simulink model "SK_x46s"  (R2026a)
settings: Solver=ode14x  StopTime=p_T  FixedStep=p_Ts
undefined symbols (not defined in the file): dspblkCoreblockFVToolHelper, gcbh, isdone_init, p_base_mass, p_base_w, p_cmd_scale, p_cost_type, p_damp_scale, p_delay_steps, p_inertia_scale, p_j6_lim, p_lambda, p_obs_mode, p_obs_noise, p_q0, p_reward_mode, p_theta, p_Ts_agent, reward_init, X, Y, Z
libraries: sm_lib x98, nesl_utility x50, rllib x1, sharedutil x1
(part 3 of 3)

== matlab function SK_x46s/Obs Transform ==
  data: u input; y output; mode input; sigma input
function y = obs_transform(u, mode, sigma)
% mode 0: Beobachtung wie im Training [ep; ev; v_base; w_base; q; dq; e_ori]
% mode 1: wie Deploy-Skript V2.1 (Befund A22): Reihenfolge [ep; ev; q; dq; v_base; w_base; e_ori],
%         Vorzeichen Soll - Ist, Basisgroessen null, e_ori = Endeffektor-Orientierung, Clipping wie V2.1
% sigma: 29x1 Standardabweichungen fuer gaussches Beobachtungsrauschen (D7), 0 = kein Rauschen.
%        Das Rauschen kommt aus MATLAB (desktop_obs_randn), damit rng-Seeds wirken.
coder.extrinsic('desktop_v21_eori', 'desktop_obs_randn');
y = u;
if any(sigma > 0)
    nz = zeros(29, 1);
    nz = desktop_obs_randn();
    y = y + sigma .* nz;
end
if mode == 1
    q = y(13:19);
    dq = y(20:26);
    e = zeros(3, 1);
    e = desktop_v21_eori(q);
    y = [-y(1:3); -y(4:6); q; dq; zeros(3, 1); zeros(3, 1); e];
    qlo = [-2*pi; -2.41; -2*pi; -2.66; -2.23; -2.01; -2*pi];
    dqlim = [1.3963; 1.3963; 1.3963; 1.3963; 1.2218; 1.2218; 1.2218];
    hi = [0.5*ones(3,1); 1.0*ones(3,1); -qlo; dqlim; 0.5*ones(3,1); 1.0*ones(3,1); pi*ones(3,1)];
    y = min(max(y, -hi), hi);
end

== matlab function SK_x46s/Reward/MATLAB Function ==
  data: ep input; reward output; ev input; dq_cmd input; dq_cmd_prev input; isDone output; w_base input; e_ori input; cost output; p_reward_mode parameter; p_base_w parameter; p_lambda parameter; p_theta parameter; p_cost_type parameter
function [reward, isDone, cost] = rewardFcn(ep, ev, dq_cmd, dq_cmd_prev, w_base, e_ori, p_reward_mode, ...
p_base_w, p_lambda, p_theta, p_cost_type)
% Reward des Tracking-Trainings mit Varianten fuer D12 (Befund A51)
%   p_reward_mode 0: wie im Training seit 09.04. (Basis-Strafen und Basis-Bonus)
%                 1: ohne Basis-Terme, wie beim fruehen PPO (Modell im Commit 50ad2ce, ohne Abbruch bei ori > 1)
%                 2: wie 0, der Basis-Bonus gilt nur bei EE-Fehler < 5 cm
%                 3: dicht und gekoppelt: glatte EE-Boni, Basis-Bonus mit der Tracking-Guete gewichtet,
%                    linearer Positionsterm -5*min(|ep|, 0,2) (hoechstens -1 pro Schritt, damit ein Abbruch
%                    nicht billiger wird als Weiterfahren). Basis-Strafen wie 0
%                 4: wie 2, dazu auf der Bahn (EE-Fehler < 5 cm) ein glatter Basis-Term
%                    +p_base_w*exp(-(ori/0,05)^2), p_base_w = 2 in D16, variiert in D17
%                 5: wie 1 (nur Tracking), dazu -p_lambda*cost (Nebenbedingung auf die Basisdrehung, X1)
%   cost: Kosten der Nebenbedingung, in allen Modi berechnet. p_cost_type 1: 1 wenn ori > p_theta,
%         2: max(0, ori - p_theta)/p_theta. In Abbruchschritten 0
mode = p_reward_mode;
cost = 0;

if any(~isfinite([ep; ev; dq_cmd; dq_cmd_prev; w_base; e_ori]))
    reward = -50;
    isDone = true;
    return;
end

dist   = norm(ep);
vel    = norm(ev);
w_norm = norm(w_base);
ori    = norm(e_ori);

if dist > 0.5 || vel > 2.0 || (mode ~= 1 && mode ~= 5 && ori > 1.0)
    reward = -50;
    isDone = true;
    return;
end

c_pos = min(ep.' * ep, 0.25);
c_vel = min(ev.' * ev, 4.0);
c_u   = min(dq_cmd.' * dq_cmd, 10.0);
du    = dq_cmd - dq_cmd_prev;
c_du  = min(du.' * du, 10.0);
c_ori = min(e_ori.' * e_ori, 0.5);
c_w   = min(w_base.' * w_base, 1.0);

if p_cost_type == 2
    cost = max(0, ori - p_theta) / p_theta;
elseif ori > p_theta
    cost = 1;
end

if mode == 1 || mode == 5
    reward = - 20.0 * c_pos - 2.0 * c_vel - 0.02 * c_u - 0.05 * c_du;
else
    reward = ...
        - 20.0  * c_pos ...
        -  2.0  * c_vel ...
        -  0.02 * c_u   ...
        -  0.05 * c_du  ...
        -  8.0  * c_ori ...
        -  4.0  * c_w;
end

if mode == 3
    g = exp(-(dist / 0.05)^2);
    reward = reward - 5.0 * min(dist, 0.2) + 1.0 * g + 3.0 * exp(-(dist / 0.02)^2) ...
        + 2.0 * g * exp(-(ori / 0.02)^2) * exp(-(w_norm / 0.01)^2);
else
    if dist < 0.05
        reward = reward + 1;
    end
    if dist < 0.02
        reward = reward + 3;
    end
    if mode == 0 && ori < 0.02 && w_norm < 0.01
        reward = reward + 2;
    end
    if mode == 2 && ori < 0.02 && w_norm < 0.01 && dist < 0.05
        reward = reward + 2;
    end
    if mode == 4 && dist < 0.05
        reward = reward + p_base_w * exp(-(ori / 0.05)^2);
        if ori < 0.02 && w_norm < 0.01
            reward = reward + 2;
        end
    end
end
if mode == 5
    reward = reward - p_lambda * cost;
end

isDone = false;
end

== matlab function SK_x46s/Robot/Impuls Monitor/MATLAB Function ==
  data: v1 input; p_tot output; w1 input; q1 input; v2 input; w2 input; q2 input; v3 input; w3 input; q3 input; v4 input; w4 input; q4 input; v5 input; w5 input; q5 input
function p_tot = totalMomentum( ...
    v1,w1,q1, ...
    v2,w2,q2, ...
    v3,w3,q3, ...
    v4,w4,q4, ...
    v5,w5,q5)

%#codegen

    % Massen
    m = [5; 1; 1; 1; 1];

    % COM-Offsets im jeweiligen Link-Frame
    r_link = [ 0.0  0.0  0.0;   % Link 1
               0.5  0.0  0.0;   % Link 2
               0.5  0.0  0.0;   % Link 3
               0.5  0.0  0.0;   % Link 4
               0.5  0.0  0.0];  % Link 5

    % Initialisiere Gesamtimpuls
    p_tot = zeros(3,1);

    % Link 1
    p_tot = p_tot + linkMomentum(v1, w1, q1, m(1), r_link(1,:).');

    % Link 2
    p_tot = p_tot + linkMomentum(v2, w2, q2, m(2), r_link(2,:).');

    % Link 3
    p_tot = p_tot + linkMomentum(v3, w3, q3, m(3), r_link(3,:).');

    % Link 4
    p_tot = p_tot + linkMomentum(v4, w4, q4, m(4), r_link(4,:).');

    % Link 5
    p_tot = p_tot + linkMomentum(v5, w5, q5, m(5), r_link(5,:).');

end

function p = linkMomentum(v, w, q, m, r_link)
% v, w: 3x1 im World-Frame
% q: 4x1 Quaternion [w x y z], Orientierung Link relativ zu World
% r_link: 3x1 COM-Offset im Link-Frame

    % COM-Offset in World-Koordinaten drehen
    r_world = quatRotate(q, r_link);

    % COM-Geschwindigkeit
    v_com = v + cross(w, r_world);

    % Impuls dieses Links
    p = m * v_com;
end

function v_out = quatRotate(q, v_in)
% rotiert v_in (3x1) mit Quaternion q = [w x y z]

    % Normalisieren zur Sicherheit
    q = q(:) / norm(q);

    w = q(1);
    x = q(2);
    y = q(3);
    z = q(4);

    % Rotationsmatrix aus Quaternion (world <- link)
    R = [1-2*(y^2+z^2),   2*(x*y - z*w),   2*(x*z + y*w);
         2*(x*y + z*w),   1-2*(x^2+z^2),   2*(y*z - x*w);
         2*(x*z - y*w),   2*(y*z + x*w),   1-2*(x^2+y^2)];

    v_out = R * v_in(:);
end

== matlab function SK_x46s/Robot/MATLAB Function2 ==
  data: q0 input; e_ori output; qb input
function e_ori = quatOriError(q0, qb)

    if qb(1) < 0, qb = -qb; end
    
    % ensure unit quaternions
    q0 = q0(:)/norm(q0); qb = qb(:)/norm(qb);
    
    % relative: q_err = conj(q0) * qb
    qconj = [ q0(1); -q0(2:4) ];
    qerr  = quatMultiply(qconj, qb);
    
    % keep scalar part non-negative to avoid flips
    if qerr(1) < 0
        qerr = -qerr;
    end
    
    w = qerr(1);
    v = qerr(2:4);
    nv = norm(v);
    
    if nv < 1e-12
        e_ori = [0;0;0];
    else
        theta = 2*atan2(nv, max(1e-12, w));
        u = v / nv;
        e_ori = theta * u;   % 3x1
    end
end

function q = quatMultiply(q1,q2)
    % [w x y z] * [w x y z]
    w1=q1(1); v1=q1(2:4); w2=q2(1); v2=q2(2:4);
    w  = w1*w2 - dot(v1,v2);
    v  = w1*v2 + w2*v1 + cross(v1,v2);
    q  = [w; v];
end
